simulink model "my_bldc_controller.before-unipolar-pwm"  (R2026a)
settings: Solver=FixedStepDiscrete  StopTime=5  FixedStep=Ts_sim
InitFcn:
  | warning('off','physmod:simscape:engine:core:advancer_errors:fallback_solve')
model workspace (MAT data in the model file):
  B_rotor = 2e-07
  C_buck = 4.7e-05
  Dmax = 0.95
  Fsw = 50000
  J_body = 0.007
  J_flywheel = 1.6e-05
  J_rotor = 5e-07
  K_A = 1
  L_buck = 0.0001
  Ts_sim = 5e-07
  Vin = 12
  f_pwm = 20000
  psi_m = 0.004
libraries: nesl_utility x18, fl_lib x16, ee_lib x13, slpidlib x2, simulink x1, eePwmGenerator x1
(part 1 of 2)
settings Model: Creator=mulusoy  LastModifiedBy=tama
settings SimscapeCC: SimscapeNominalValues="[{\"value\":\"1\",\"unit\":\"A\"},{\"value\":\"1\",\"unit\":\"bar\"},{\"value\":\"1\",\"unit\":\"cm^2\"},{\"value\":\"1\",\"unit\":\"cm^3/s\"},{\"value\":\"1\",\"unit\":\"kJ/kg\"},{\"value\":\"1\",\"unit\":\"kW\"},{\"value\":\"1\",\"unit\":\"l\"},{\"value\":\"1\",\"unit\":\"N\"},{\"value\":\"1\",\"unit\":\"N*m\"},{\"value\":\"1\",\"unit\":\"V\"}]"  SimscapeLogType=none  SimscapeLogDataHistory=5000.0

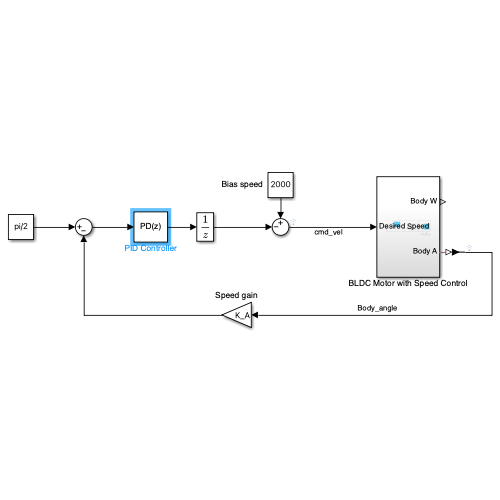
[thumbnail: Simulink's stored preview of the top-level diagram]
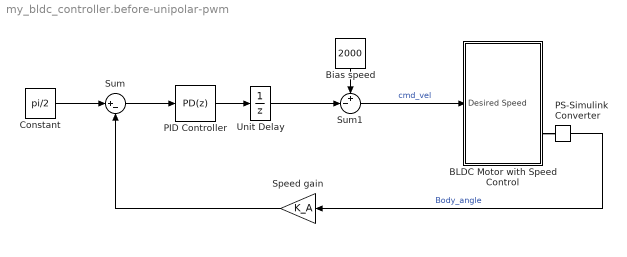
== system my_bldc_controller.before-unipolar-pwm ==
  BLDC Motor with Speed Control : Subsystem
  Bias speed : Constant  Value=2000
  Constant : Constant  Value=pi/2
  PID Controller : slpidlib/PID Controller  Controller=PD  Form=Parallel  TimeDomain=Discrete-time  UseExternalTs=off  SampleTime=0.01  IntegratorMethod=Forward Euler  FilterMethod=Forward Euler  ControllerParametersSource=internal  P=3500  I=1  UseKiTs=off  D=0  UseExternalDerivativeSource=off  N=100  UseFilter=on  TunerSelectOption=Transfer Function Based (PID Tuner App)  InitialConditionSource=internal  InitialConditionForIntegrator=0  InitialConditionForFilter=0  DifferentiatorICPrevScaledInput=0  ExternalReset=none  TrackingMode=off  Kt=1  LimitOutput=off  SatLimitsSource=internal  UpperSaturationLimit=inf  LowerSaturationLimit=-inf  LinearizeAsGain=on  AntiWindupMode=clamping  Kb=1  LimitIntegrator=off  UpperIntegratorSaturationLimit=inf  LowerIntegratorSaturationLimit=-inf  POutMin=[]  POutMax=[]  IOutMin=[]  IOutMax=[]  DOutMin=[]  DOutMax=[]  NOutMin=[]  NOutMax=[]  SumOutMin=[]  SumOutMax=[]  SaturationOutMin=[]  SaturationOutMax=[]  PParamMin=[]  PParamMax=[]  IParamMin=[]  IParamMax=[]  DParamMin=[]  DParamMax=[]  NParamMin=[]  NParamMax=[]  KbParamMin=[]  KbParamMax=[]  KtParamMin=[]  KtParamMax=[]  KbOutMin=[]  KbOutMax=[]  KtOutMin=[]  KtOutMax=[]  IntegratorOutMin=[]  IntegratorOutMax=[]  FilterOutMin=[]  FilterOutMax=[]  SumI1OutMin=[]  SumI1OutMax=[]  SumI2OutMin=[]  SumI2OutMax=[]  SumI3OutMin=[]  SumI3OutMax=[]  SumI4OutMin=[]  SumI4OutMax=[]  SumDOutMin=[]  SumDOutMax=[]  DifferentiatorOutMin=[]  DifferentiatorOutMax=[]  FilterDiffOutCoefMin=[]  FilterDiffOutCoefMax=[]  ReciprocalOutMin=[]  ReciprocalOutMax=[]  SumDenOutMin=[]  SumDenOutMax=[]  SumNumOutMin=[]  SumNumOutMax=[]  DivideOutMin=[]  DivideOutMax=[]  UdiffTsProdOutMin=[]  UdiffTsProdOutMax=[]  NTsProdOutMin=[]  NTsProdOutMax=[]  UintegralTsProdOutMin=[]  UintegralTsProdOutMax=[]  UngainTsProdOutMin=[]  UngainTsProdOutMax=[]  ClampingZeroOutDataTypeStr=Inherit: Inherit via back propagation  ClampingZeroOutMin=[]  ClampingZeroOutMax=[]  FilterDenConstantOutDataTypeStr=Inherit: Inherit via back propagation  FilterDenConstantOutMin=[]  FilterDenConstantOutMax=[]  PCopyOutDataTypeStr=Inherit: Inherit via back propagation  PCopyOutMin=[]  PCopyOutMax=[]  NCopyOutDataTypeStr=Inherit: Inherit via back propagation  NCopyOutMin=[]  NCopyOutMax=[]  IntegratorContinuousStateAttributes=''  IntegratorStateMustResolveToSignalObject=off  IntegratorRTWStateStorageClass=Auto  FilterContinuousStateAttributes=''  FilterStateMustResolveToSignalObject=off  FilterRTWStateStorageClass=Auto  ParallelPVariant=InternalParameters  IdealPVariant=Disabled  IVariant=Disabled  DVariant=InternalParameters  IntegratorVariant=Disabled  SatVariant=Disabled  AWVariant=Disabled  PCopyVariant=Disabled  TRVariant=Disabled  FdbkBlocksVariant=Forward  IdealPFdbkVariant=Disabled  SatFdbkVariant=Disabled  DerivativeFilterVariant=ForwardEulerFilter  NVariant=InternalParameters  NCopyVariant=Disabled  FilterICVariant=InternalICsFilter  IntegratorICVariant=Disabled  ExternalResetVariant=Disabled  TRSumVariant=Passthrough  SumFdbkVariant=Disabled  SumVariant=Sum_PD  TsampFilterVariant=InternalTs  TsampNgainVariant=Passthrough  TsampIntegralVariant=Disabled_SignalSpec  ExternalSaturationOutDataTypeStr=Inherit: Same as second input  DerivativeSourceVariant=ErrorSignal  PreIntVariant=InternalPreInt
  PS-Simulink Converter : nesl_utility/PS-Simulink Converter  PhysicalDomain=network_engine_domain  SubClassName=ps_output  LeftPortType=input  RightPortType=output  PseudoPeriodic=off  Frequencies=[]  VectorFormat=inherit  Unit=inherit  AffineConversion=off
  Speed gain : Gain  Gain=K_A
  Sum : Sum  Inputs=|+-
  Sum1 : Sum  Inputs=+-|
  Unit Delay : UnitDelay  SampleTime=-1
  wires:
  PID Controller/1 -> Unit Delay/1
  PS-Simulink Converter/1 -> Speed gain/1  "Body_angle"
  Constant/1 -> Sum/1
  Sum/1 -> PID Controller/1
  Speed gain/1 -> Sum/2
  Bias speed/1 -> Sum1/1
  Unit Delay/1 -> Sum1/2
  Sum1/1 -> BLDC Motor with Speed Control/1(Desired Speed)  "cmd_vel"
  connections:
  BLDC Motor with Speed Control/RConn2 -- PS-Simulink Converter/LConn1

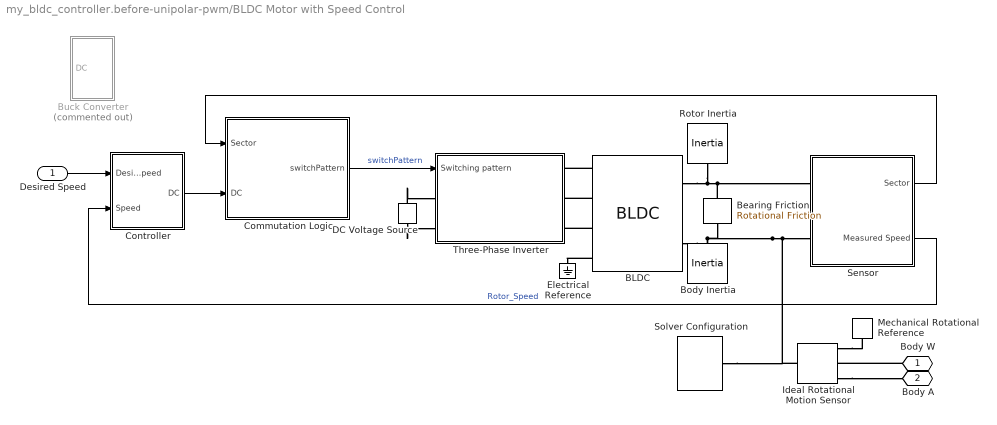
== system my_bldc_controller.before-unipolar-pwm/BLDC Motor with Speed Control ==
  Desired Speed : Inport
  BLDC : ee_lib/Electromechanical/Permanent Magnet/BLDC  port_option=ee.enum.threePhasePort.expanded  rotor_param=1  pm_flux_linkage=psi_m Wb  theta_constant=120/1 deg  emf_max=9.6 V  w_meas=600 rpm  DphiDtheta_tab=[0, -.1528, -.1528, .1528, .1528, 0] Wb/rad  back_emf_tab=[0, -9.6, -9.6, 9.6, 9.6, 0] V  rotor_angle_tab=[0, 7.5, 22.5, 37.5, 52.5, 60] deg  nPolePairs=1  axes_param=2  winding_type=ee.enum.statorconnection.wye  stator_param=ee.enum.statorparam.LdLqL0  machine_param=ee.enum.dqparameterization.constant  Ld=0.2 mH  Lq=0.2 mH  idVec=[-200, 0, 200] A  iqVec=[-200, 0, 200] A  LdMatrix=0.00022 * ones(3, 3) H  LqMatrix=0.00022 * ones(3, 3) H  L0=0.2 mH  Ls=0.0002 H  Lm=0 H  Ms=0.00002 H  Rs=2 Ohm  zero_sequence=ee.enum.park.zerosequence.include  loss_param=ee.enum.ironloss.none  losses_oc=[0, 0, 0] W  losses_sc=[0, 0, 0] W  f_losses=60 Hz  Isc_losses=95 A  J=J_rotor kg*m^2  lam=B_rotor N*m/(rad/s)  i_d_specify=off  i_d_priority=None  i_d=0 A  i_d_nominal_specify=off  i_d_nominal_value=1  i_d_nominal_unit=A  i_q_specify=off  i_q_priority=None  i_q=0 A  i_q_nominal_specify=off  i_q_nominal_value=1  i_q_nominal_unit=A  torque_specify=off  torque_priority=None  torque=0 N*m  torque_nominal_specify=off  torque_nominal_value=1  torque_nominal_unit=N*m  angular_velocity_specify=on  angular_velocity_priority=High  angular_velocity=2000 rpm  angular_velocity_nominal_specify=off  angular_velocity_nominal_value=1  angular_velocity_nominal_unit=rpm  angular_position_specify=off  angular_position_priority=High  angular_position=0 deg  angular_position_nominal_specify=off  angular_position_nominal_value=1  angular_position_nominal_unit=deg  alpha=3.93e-3 1/K  alpha_flux=-0.001 1/K  Tmeas=298.15 K  stator_thermal_mass=100 J/K  rotor_thermal_mass=200 J/K  Rm_percent_rotor=90  Rd_percent_rotor=30  temperatureA_specify=off  temperatureA_priority=High  temperatureA=25 degC  temperatureA_nominal_specify=off  temperatureA_nominal_value=1  temperatureA_nominal_unit=degC  temperatureB_specify=off  temperatureB_priority=High  temperatureB=25 degC  temperatureB_nominal_specify=off  temperatureB_nominal_value=1  temperatureB_nominal_unit=degC  temperatureC_specify=off  temperatureC_priority=High  temperatureC=25 degC  temperatureC_nominal_specify=off  temperatureC_nominal_value=1  temperatureC_nominal_unit=degC  temperatureR_specify=off  temperatureR_priority=High  temperatureR=25 degC  temperatureR_nominal_specify=off  temperatureR_nominal_value=1  temperatureR_nominal_unit=degC
  Bearing Friction : fl_lib/Mechanical/Rotational Elements/Rotational Friction  brkwy_trq=0.05 m*mN  brkwy_vel=0.1 rad/s  Col_trq=0.05 m*mN  visc_coef=0 N*m*s/rad  w_specify=off  w_priority=None  w=0 rad/s  w_nominal_specify=off  w_nominal_value=1  w_nominal_unit=rad/s  t_specify=off  t_priority=None  t=0 N*m  t_nominal_specify=off  t_nominal_value=1  t_nominal_unit=N*m
  Body Inertia : fl_lib/Mechanical/Rotational Elements/Inertia  inertia=J_body kg*m^2  num_ports=foundation.enum.numPorts2.one  w_specify=on  w_priority=High  w=0 rad/s  w_nominal_specify=off  w_nominal_value=1  w_nominal_unit=rad/s  t_specify=off  t_priority=None  t=0 N*m  t_nominal_specify=off  t_nominal_value=1  t_nominal_unit=N*m
  Buck Converter : Subsystem  Description=Label-mode variant. Averaged (default): Vin*d controlled source + L/C filter, run with Ts_sim = 1e-5. Switching: PWM + MOSFETs at Fsw, needs Ts_sim <= 2e-7 (1% duty resolution at 50 kHz) - set Ts_sim in the model workspace before switching.  Commented=on  Variant=on  VariantControlMode=label  LabelModeActiveChoice=Averaged
  Commutation Logic : Subsystem
  Controller : Subsystem
  DC Voltage Source : ee_lib/Additional Components/SPICE Sources/DC Voltage Source  DC=12 V
  Electrical Reference : fl_lib/Electrical/Electrical Elements/Electrical Reference
  Ideal Rotational Motion Sensor : fl_lib/Mechanical/Mechanical Sensors/Ideal Rotational Motion Sensor  reference=foundation.enum.MeasurementReference.difference  acceleration_port=false  velocity_port=true  position_port=true  wrap_angle=false  offset=0 rad
  Mechanical Rotational Reference : fl_lib/Mechanical/Rotational Elements/Mechanical Rotational Reference
  Rotor Inertia : fl_lib/Mechanical/Rotational Elements/Inertia  inertia=J_flywheel kg*m^2  num_ports=foundation.enum.numPorts2.one  w_specify=on  w_priority=High  w=2000 rpm  w_nominal_specify=off  w_nominal_value=1  w_nominal_unit=rad/s  t_specify=off  t_priority=None  t=0 N*m  t_nominal_specify=off  t_nominal_value=1  t_nominal_unit=N*m
  Sensor : Subsystem
  Solver Configuration : nesl_utility/Solver Configuration  PhysicalDomain=network_engine_domain  SubClassName=solver  LeftPortType=input  RightPortType=generic  Tones=[]  Harmonics=[]  SimulateNoise=off  Profile=off  UseLocalSampling=off  EnableSwitchedLinearOptims=on  FrequencyDomain=off  UseCCode=off  RelTol=0.001  AbsTol=1e-06  MinStep=1e-09  ToWorkspace=off  RevertToSquareIcSolve=off  NumHomotopyIterations=100  PhasorMode=off  PhasorModeNumHarmonics=1  ConsistencySolver=NEWTON_FTOL  CanonicalOrdering=UNORDERED  OptimizeIntermediates=UNOPTIMIZED  IndexReductionMethod=DerivativeReplacement  DoDC=off  ResidualTolerance=1e-09  ConsistencyTolSource=GLOBAL  ConsistencyAbsTol=0.001  ConsistencyRelTol=0.001  ConsistencyTolFactor=0.001  UseLocalSolver=on  LocalSolverChoice=NE_BACKWARD_EULER_ADVANCER  ResolveIndetEquations=on  FunctionEvalNumThread=1  LocalSolverSampleTime=Ts_sim  DoFixedCost=on  MaxNonlinIter=4  MaxModeIter=2  ComputeImpulses=off  ImpulseIterations=2  LinearAlgebra=auto  LinearAlgebraNumThread=0  EquationFormulation=NE_TIME_EF  DelaysMemoryBudget=1024  AutomaticFiltering=off  FilteringTimeConstant=0.001  PartitionStorageMethod=AS_NEEDED  PartitionMemoryBudget=1024  PartitionMethod=ROBUST  MultibodyUseLocalSolver=off  MultibodyLocalSolverChoice=ODE1  MultibodyLocalSolverSampleTime=0.001
  Three-Phase Inverter : Subsystem
  Body W : PMIOPort  Side=Right
  Body A : PMIOPort  Port=2  Side=Right
  wires:
  Commutation Logic/1(switchPattern) -> Three-Phase Inverter/1(Switching pattern)  "switchPattern"
  Sensor/2(Measured Speed) -> Controller/2(Speed)  "Rotor_Speed"
  Sensor/1(Sector) -> Commutation Logic/1(Sector)
  Controller/1(DC) -> Commutation Logic/2(DC)
  Desired Speed/1 -> Controller/1(Desired Speed)
  connections:
  BLDC/LConn2 -- Three-Phase Inverter/RConn2
  BLDC/LConn1 -- Three-Phase Inverter/RConn1
  BLDC/LConn4 -- Electrical Reference/LConn1
  BLDC/LConn3 -- Three-Phase Inverter/RConn3
  Ideal Rotational Motion Sensor/RConn1 -- Mechanical Rotational Reference/LConn1
  Body W/RConn1 -- Ideal Rotational Motion Sensor/RConn2
  Ideal Rotational Motion Sensor/RConn3 -- Body A/RConn1
  BLDC/RConn2 -- Bearing Friction/RConn1 -- Solver Configuration/RConn1 -- Ideal Rotational Motion Sensor/LConn1 -- Sensor/LConn2 -- Body Inertia/LConn1
  BLDC/RConn1 -- Rotor Inertia/LConn1 -- Bearing Friction/LConn1 -- Sensor/LConn1
  DC Voltage Source/LConn1 -- Three-Phase Inverter/LConn1
  DC Voltage Source/RConn1 -- Three-Phase Inverter/LConn2

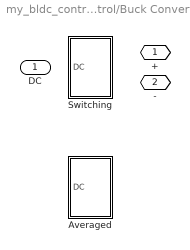
== system my_bldc_controller.before-unipolar-pwm/BLDC Motor with Speed Control/Buck Converter ==
  DC : Inport
  Averaged : Subsystem  VariantControl=Averaged
  Switching : Subsystem  VariantControl=Switching
  + : PMIOPort  Side=Right
  - : PMIOPort  Port=2  Side=Right

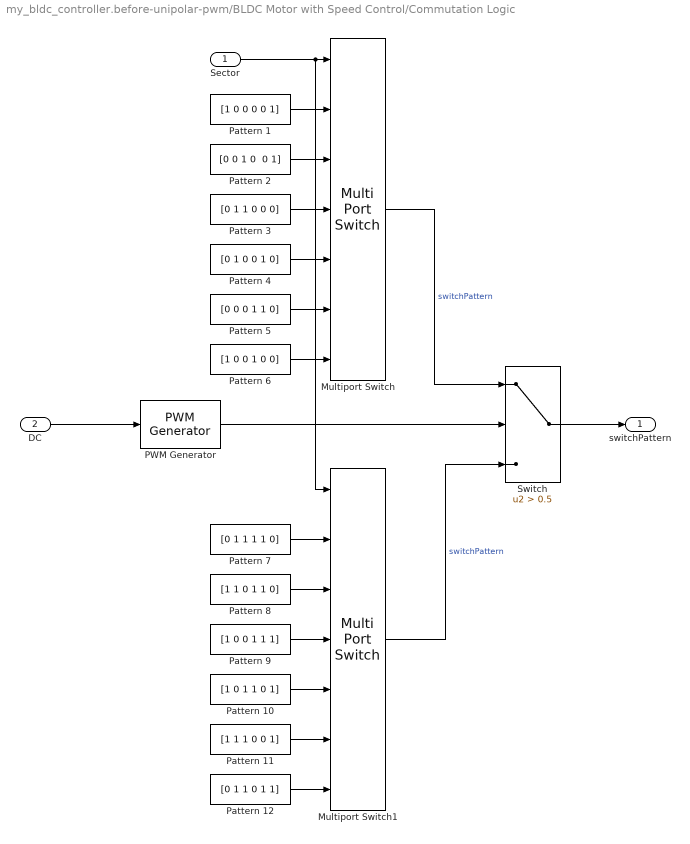
== system my_bldc_controller.before-unipolar-pwm/BLDC Motor with Speed Control/Commutation Logic ==
  Sector : Inport
  DC : Inport  Port=2
  Multiport Switch : MultiPortSwitch  Inputs=6  SaturateOnIntegerOverflow=off  InputSameDT=off
  Multiport Switch1 : MultiPortSwitch  Inputs=6  SaturateOnIntegerOverflow=off  InputSameDT=off
  PWM Generator : eePwmGenerator/PWM Generator  CarrCount=Up  Tper=1/f_pwm  Tdelay=0  Ts=5e-5
  Pattern 1 : Constant  Value=[1 0 0 0 0 1]
  Pattern 10 : Constant  Value=[1 0 1 1 0 1]
  Pattern 11 : Constant  Value=[1 1 1 0 0 1]
  Pattern 12 : Constant  Value=[0 1 1 0 1 1]
  Pattern 2 : Constant  Value="[0 0 1 0  0 1]"
  Pattern 3 : Constant  Value=[0 1 1 0 0 0]
  Pattern 4 : Constant  Value=[0 1 0 0 1 0]
  Pattern 5 : Constant  Value=[0 0 0 1 1 0]
  Pattern 6 : Constant  Value=[1 0 0 1 0 0]
  Pattern 7 : Constant  Value=[0 1 1 1 1 0]
  Pattern 8 : Constant  Value=[1 1 0 1 1 0]
  Pattern 9 : Constant  Value=[1 0 0 1 1 1]
  Switch : Switch  Criteria=u2 > Threshold  Threshold=0.5  SaturateOnIntegerOverflow=off  InputSameDT=off
  switchPattern : Outport
  wires:
  Pattern 3/1 -> Multiport Switch/4
  Pattern 5/1 -> Multiport Switch/6
  Pattern 2/1 -> Multiport Switch/3
  Pattern 4/1 -> Multiport Switch/5
  Multiport Switch/1 -> Switch/1  "switchPattern"
  Pattern 6/1 -> Multiport Switch/7
  Pattern 1/1 -> Multiport Switch/2
  Sector/1 -> Multiport Switch1/1, Multiport Switch/1
  Pattern 7/1 -> Multiport Switch1/2
  Pattern 12/1 -> Multiport Switch1/7
  Pattern 10/1 -> Multiport Switch1/5
  Pattern 8/1 -> Multiport Switch1/3
  Pattern 11/1 -> Multiport Switch1/6
  Pattern 9/1 -> Multiport Switch1/4
  DC/1 -> PWM Generator/1
  Multiport Switch1/1 -> Switch/3  "switchPattern"
  Switch/1 -> switchPattern/1
  PWM Generator/1 -> Switch/2

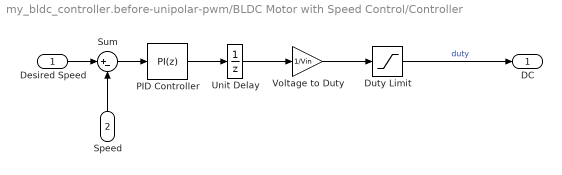
== system my_bldc_controller.before-unipolar-pwm/BLDC Motor with Speed Control/Controller ==
  Desired Speed : Inport
  Speed : Inport  Port=2
  Duty Limit : Saturate  UpperLimit=Dmax  LowerLimit=0
  PID Controller : slpidlib/PID Controller  Controller=PI  Form=Parallel  TimeDomain=Discrete-time  UseExternalTs=off  SampleTime=1e-5  IntegratorMethod=Forward Euler  FilterMethod=Forward Euler  ControllerParametersSource=internal  P=0.06188  I=2.149  UseKiTs=off  D=0  UseExternalDerivativeSource=off  N=100  UseFilter=on  TunerSelectOption=Transfer Function Based (PID Tuner App)  InitialConditionSource=internal  InitialConditionForIntegrator=0  InitialConditionForFilter=0  DifferentiatorICPrevScaledInput=0  ExternalReset=none  TrackingMode=off  Kt=1  LimitOutput=on  SatLimitsSource=internal  UpperSaturationLimit=Dmax*Vin  LowerSaturationLimit=0  LinearizeAsGain=on  AntiWindupMode=clamping  Kb=1  LimitIntegrator=off  UpperIntegratorSaturationLimit=inf  LowerIntegratorSaturationLimit=-inf  POutMin=[]  POutMax=[]  IOutMin=[]  IOutMax=[]  DOutMin=[]  DOutMax=[]  NOutMin=[]  NOutMax=[]  SumOutMin=[]  SumOutMax=[]  SaturationOutMin=[]  SaturationOutMax=[]  PParamMin=[]  PParamMax=[]  IParamMin=[]  IParamMax=[]  DParamMin=[]  DParamMax=[]  NParamMin=[]  NParamMax=[]  KbParamMin=[]  KbParamMax=[]  KtParamMin=[]  KtParamMax=[]  KbOutMin=[]  KbOutMax=[]  KtOutMin=[]  KtOutMax=[]  IntegratorOutMin=[]  IntegratorOutMax=[]  FilterOutMin=[]  FilterOutMax=[]  SumI1OutMin=[]  SumI1OutMax=[]  SumI2OutMin=[]  SumI2OutMax=[]  SumI3OutMin=[]  SumI3OutMax=[]  SumI4OutMin=[]  SumI4OutMax=[]  SumDOutMin=[]  SumDOutMax=[]  DifferentiatorOutMin=[]  DifferentiatorOutMax=[]  FilterDiffOutCoefMin=[]  FilterDiffOutCoefMax=[]  ReciprocalOutMin=[]  ReciprocalOutMax=[]  SumDenOutMin=[]  SumDenOutMax=[]  SumNumOutMin=[]  SumNumOutMax=[]  DivideOutMin=[]  DivideOutMax=[]  UdiffTsProdOutMin=[]  UdiffTsProdOutMax=[]  NTsProdOutMin=[]  NTsProdOutMax=[]  UintegralTsProdOutMin=[]  UintegralTsProdOutMax=[]  UngainTsProdOutMin=[]  UngainTsProdOutMax=[]  ClampingZeroOutDataTypeStr=Inherit: Inherit via back propagation  ClampingZeroOutMin=[]  ClampingZeroOutMax=[]  FilterDenConstantOutDataTypeStr=Inherit: Inherit via back propagation  FilterDenConstantOutMin=[]  FilterDenConstantOutMax=[]  PCopyOutDataTypeStr=Inherit: Inherit via back propagation  PCopyOutMin=[]  PCopyOutMax=[]  NCopyOutDataTypeStr=Inherit: Inherit via back propagation  NCopyOutMin=[]  NCopyOutMax=[]  IntegratorContinuousStateAttributes=''  IntegratorStateMustResolveToSignalObject=off  IntegratorRTWStateStorageClass=Auto  FilterContinuousStateAttributes=''  FilterStateMustResolveToSignalObject=off  FilterRTWStateStorageClass=Auto  ParallelPVariant=InternalParameters  IdealPVariant=Disabled  IVariant=InternalParameters  DVariant=Disabled  IntegratorVariant=Discrete  SatVariant=Enabled  AWVariant=DiscClampingParallel  PCopyVariant=Disabled  TRVariant=Disabled  FdbkBlocksVariant=Forward  IdealPFdbkVariant=Disabled  SatFdbkVariant=Disabled  DerivativeFilterVariant=Disabled  NVariant=Disabled  NCopyVariant=Disabled_SignalSpec  FilterICVariant=Disabled  IntegratorICVariant=InternalICs  ExternalResetVariant=Disabled  TRSumVariant=Passthrough  SumFdbkVariant=Disabled  SumVariant=Sum_PI  TsampFilterVariant=InternalTs  TsampNgainVariant=Passthrough  TsampIntegralVariant=Disabled_SignalSpec  ExternalSaturationOutDataTypeStr=Inherit: Same as second input  DerivativeSourceVariant=Disabled  PreIntVariant=InternalPreInt
  Sum : Sum  Inputs=|+-
  Unit Delay : UnitDelay  SampleTime=-1
  Voltage to Duty : Gain  Gain=1/Vin
  DC : Outport
  wires:
  Duty Limit/1 -> DC/1  "duty"
  Unit Delay/1 -> Voltage to Duty/1
  Speed/1 -> Sum/2
  Sum/1 -> PID Controller/1
  Voltage to Duty/1 -> Duty Limit/1
  Desired Speed/1 -> Sum/1
  PID Controller/1 -> Unit Delay/1

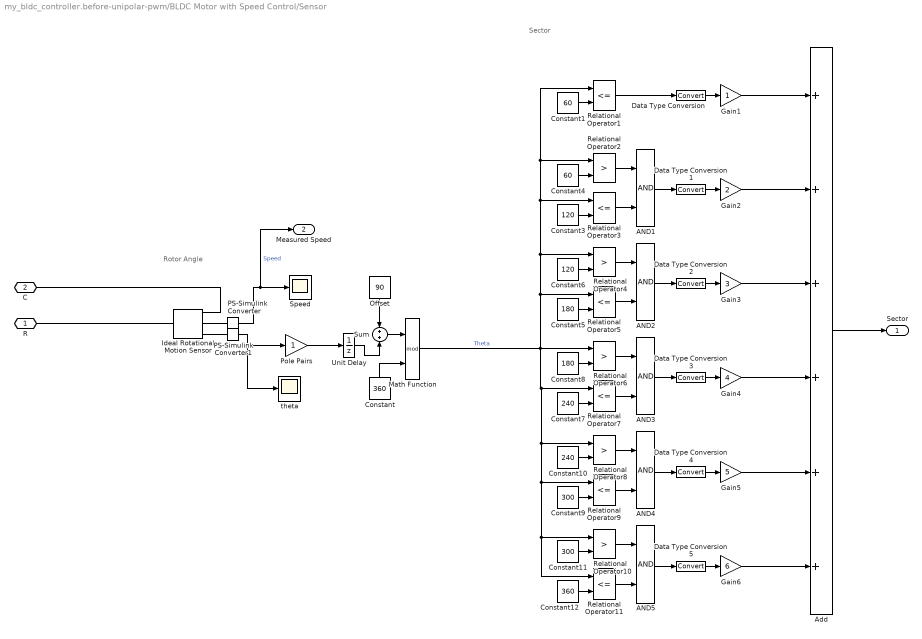
== system my_bldc_controller.before-unipolar-pwm/BLDC Motor with Speed Control/Sensor ==
  note: Rotor Angle
  note: Sector
  AND{1..5} (5 alike) : Logic  AllPortsSameDT=off  OutDataTypeStr=boolean
  Add : Sum  Inputs=6
  Constant : Constant  Value=360
  Constant1 : Constant  Value=60
  Constant10 : Constant  Value=240
  Constant11 : Constant  Value=300
  Constant12 : Constant  Value=360
  Constant3 : Constant  Value=120
  Constant4 : Constant  Value=60
  Constant5 : Constant  Value=180
  Constant6 : Constant  Value=120
  Constant7 : Constant  Value=240
  Constant8 : Constant  Value=180
  Constant9 : Constant  Value=300
  Data Type Conversion{,1..5} (6 alike) : DataTypeConversion  SaturateOnIntegerOverflow=off  RndMeth=Floor
  Gain1 : Gain
  Gain2 : Gain  Gain=2
  Gain3 : Gain  Gain=3
  Gain4 : Gain  Gain=4
  Gain5 : Gain  Gain=5
  Gain6 : Gain  Gain=6
  Ideal Rotational Motion Sensor : fl_lib/Mechanical/Mechanical Sensors/Ideal Rotational Motion Sensor  reference=foundation.enum.MeasurementReference.difference  acceleration_port=false  velocity_port=true  position_port=true  wrap_angle=false  offset=0 deg
  Math Function : Math  Operator=mod
  Offset : Constant  Value=90
  PS-Simulink Converter : nesl_utility/PS-Simulink Converter  PhysicalDomain=network_engine_domain  SubClassName=ps_output  LeftPortType=input  RightPortType=output  PseudoPeriodic=off  Frequencies=[]  VectorFormat=1-D array  Unit=rpm  AffineConversion=off
  PS-Simulink Converter1 : nesl_utility/PS-Simulink Converter  PhysicalDomain=network_engine_domain  SubClassName=ps_output  LeftPortType=input  RightPortType=output  PseudoPeriodic=off  Frequencies=[]  VectorFormat=1-D array  Unit=deg  AffineConversion=off
  Pole Pairs : Gain
  Relational Operator{1,3,5,7,9,11} (6 alike) : RelationalOperator  Operator=<=  OutDataTypeStr=boolean  RndMeth=Simplest  InputSameDT=off
  Relational Operator{2,4,6,8,10} (5 alike) : RelationalOperator  Operator=>  OutDataTypeStr=boolean  RndMeth=Simplest  InputSameDT=off
  Speed : Scope
      settings: ActiveDisplayYMinimum=-51.95479  ActiveDisplayYMaximum=223.68655  DataLoggingVariableName=theta
  Sum : Sum  Inputs=+|+
  Unit Delay : UnitDelay  SampleTime=-1
  theta : Scope
      settings: ActiveDisplayYMinimum=-1  ActiveDisplayYMaximum=1  DataLoggingVariableName=ScopeData2
  R : PMIOPort  Side=Left
  C : PMIOPort  Port=2  Side=Left
  Sector : Outport
  Measured Speed : Outport  Port=2
  wires:
  Add/1 -> Sector/1
  Gain6/1 -> Add/6
  Gain5/1 -> Add/5
  Gain4/1 -> Add/4
  Gain3/1 -> Add/3
  Gain2/1 -> Add/2
  Gain1/1 -> Add/1
  Relational Operator5/1 -> AND2/2
  Relational Operator10/1 -> AND5/1
  AND1/1 -> Data Type Conversion1/1
  Constant11/1 -> Relational Operator10/2
  AND5/1 -> Data Type Conversion5/1
  Constant12/1 -> Relational Operator11/2
  Data Type Conversion/1 -> Gain1/1
  AND2/1 -> Data Type Conversion2/1
  Relational Operator1/1 -> Data Type Conversion/1
  Data Type Conversion2/1 -> Gain3/1
  Data Type Conversion1/1 -> Gain2/1
  Data Type Conversion5/1 -> Gain6/1
  AND3/1 -> Data Type Conversion3/1
  Constant8/1 -> Relational Operator6/2
  Constant7/1 -> Relational Operator7/2
  Relational Operator6/1 -> AND3/1
  Data Type Conversion4/1 -> Gain5/1
  Relational Operator2/1 -> AND1/1
  AND4/1 -> Data Type Conversion4/1
  Relational Operator9/1 -> AND4/2
  Constant5/1 -> Relational Operator5/2
  Relational Operator3/1 -> AND1/2
  Constant3/1 -> Relational Operator3/2
  Relational Operator7/1 -> AND3/2
  Relational Operator4/1 -> AND2/1
  Constant4/1 -> Relational Operator2/2
  Constant1/1 -> Relational Operator1/2
  Data Type Conversion3/1 -> Gain4/1
  Relational Operator8/1 -> AND4/1
  Constant10/1 -> Relational Operator8/2
  Constant6/1 -> Relational Operator4/2
  Constant9/1 -> Relational Operator9/2
  Relational Operator11/1 -> AND5/2
  Math Function/1 -> Relational Operator6/1, Relational Operator1/1, Relational Operator2/1, Relational Operator3/1, Relational Operator4/1, Relational Operator5/1, Relational Operator7/1, Relational Operator8/1, Relational Operator10/1, Relational Operator11/1, Relational Operator9/1  "Theta"
  Pole Pairs/1 -> Unit Delay/1
  PS-Simulink Converter1/1 -> theta/1, Pole Pairs/1
  PS-Simulink Converter/1 -> Measured Speed/1, Speed/1  "Speed"
  Constant/1 -> Math Function/2
  Unit Delay/1 -> Sum/2
  Offset/1 -> Sum/1
  Sum/1 -> Math Function/1
  connections:
  Ideal Rotational Motion Sensor/LConn1 -- R/RConn1
  PS-Simulink Converter/LConn1 -- Ideal Rotational Motion Sensor/RConn2
  Ideal Rotational Motion Sensor/RConn1 -- C/RConn1
  Ideal Rotational Motion Sensor/RConn3 -- PS-Simulink Converter1/LConn1
